simulink model "all_sc_0001_0193"  (R2026a)
settings: Solver=VariableStepAuto  StopTime=40  FixedStep=0.1  MaxStep=.1
model workspace (MAT data in the model file):
  T = [0 0.05 0.1 0.15 0.2 0.25 0.3 0.35 0.4 0.45 0.5 0.55 ... (701 elements, 701x1)]
  U = [3.99594136536 3.99594136536 3.99594136536 3.99594136536 3.99594136536 3.99594136536 3.99594136536 3.99594136536 3.99594136536 3.99594136536 3.99594136536 3.99594136536 ... (701 elements, 701x1)]
undefined symbols (not defined in the file): A, B, C, Dd
(part 2 of 3)

== system all_sc_0001_0193/Subsystem/Steam Condenser1/FIMWB_011 ==
  Original : Inport
  Result : Outport
  wires:
  Original/1 -> Result/1

== system all_sc_0001_0193/Subsystem/Steam Condenser1/FIMWB_012 ==
  Original : Inport
  Result : Outport
  wires:
  Original/1 -> Result/1

== system all_sc_0001_0193/Subsystem/Steam Condenser1/FIMWB_013 ==
  Original : Inport
  Result : Outport
  wires:
  Original/1 -> Result/1

== system all_sc_0001_0193/Subsystem/Steam Condenser1/FIMWB_014 ==
  Original : Inport
  Result : Outport
  wires:
  Original/1 -> Result/1

== system all_sc_0001_0193/Subsystem/Steam Condenser1/FIMWB_015 ==
  Original : Inport
  Result : Outport
  wires:
  Original/1 -> Result/1

== system all_sc_0001_0193/Subsystem/Steam Condenser1/FIMWB_016 ==
  Original : Inport
  Result : Outport
  wires:
  Original/1 -> Result/1

== system all_sc_0001_0193/Subsystem/Steam Condenser1/FIMWB_017 ==
  Original : Inport
  Result : Outport
  wires:
  Original/1 -> Result/1

== system all_sc_0001_0193/Subsystem/Steam Condenser1/FIMWB_018 ==
  Original : Inport
  Result : Outport
  wires:
  Original/1 -> Result/1

== system all_sc_0001_0193/Subsystem/Steam Condenser1/FIMWB_019 ==
  Original : Inport
  Result : Outport
  wires:
  Original/1 -> Result/1

== system all_sc_0001_0193/Subsystem/Steam Condenser1/FIMWB_020 ==
  Original : Inport
  Result : Outport
  wires:
  Original/1 -> Result/1

== system all_sc_0001_0193/Subsystem/Steam Condenser1/FIMWB_021 ==
  Original : Inport
  Result : Outport
  wires:
  Original/1 -> Result/1

== system all_sc_0001_0193/Subsystem/Steam Condenser1/FIMWB_022 ==
  Original : Inport
  Result : Outport
  wires:
  Original/1 -> Result/1

== system all_sc_0001_0193/Subsystem/Steam Condenser1/FIMWB_023 ==
  Original : Inport
  Result : Outport
  wires:
  Original/1 -> Result/1

== system all_sc_0001_0193/Subsystem/Steam Condenser1/FIMWB_024 ==
  Original : Inport
  Result : Outport
  wires:
  Original/1 -> Result/1

== system all_sc_0001_0193/Subsystem/Steam Condenser1/FIMWB_025 ==
  Original : Inport
  Result : Outport
  wires:
  Original/1 -> Result/1

== system all_sc_0001_0193/Subsystem/Steam Condenser1/FIMWB_026 ==
  Original : Inport
  Result : Outport
  wires:
  Original/1 -> Result/1

== system all_sc_0001_0193/Subsystem/Steam Condenser1/FIMWB_027 ==
  Original : Inport
  Result : Outport
  wires:
  Original/1 -> Result/1

== system all_sc_0001_0193/Subsystem/Steam Condenser1/FIMWB_028 ==
  Original : Inport
  Result : Outport
  wires:
  Original/1 -> Result/1

== system all_sc_0001_0193/Subsystem/Steam Condenser1/FIMWB_029 ==
  Original : Inport
  Result : Outport
  wires:
  Original/1 -> Result/1

== system all_sc_0001_0193/Subsystem/Steam Condenser1/FIMWB_030 ==
  Original : Inport
  Result : Outport
  wires:
  Original/1 -> Result/1

== system all_sc_0001_0193/Subsystem/Steam Condenser1/FIMWB_031 ==
  Original : Inport
  Result : Outport
  wires:
  Original/1 -> Result/1

== system all_sc_0001_0193/Subsystem/Steam Condenser1/FIMWB_032 ==
  Original : Inport
  Result : Outport
  wires:
  Original/1 -> Result/1

== system all_sc_0001_0193/Subsystem/Steam Condenser1/FIMWB_033 ==
  Original : Inport
  Result : Outport
  wires:
  Original/1 -> Result/1

== system all_sc_0001_0193/Subsystem/Steam Condenser1/FIMWB_034 ==
  Original : Inport
  Result : Outport
  wires:
  Original/1 -> Result/1

== system all_sc_0001_0193/Subsystem/Steam Condenser1/FIMWB_035 ==
  Original : Inport
  Result : Outport
  wires:
  Original/1 -> Result/1

== system all_sc_0001_0193/Subsystem/Steam Condenser1/FIMWB_036 ==
  Original : Inport
  Result : Outport
  wires:
  Original/1 -> Result/1

== system all_sc_0001_0193/Subsystem/Steam Condenser1/FIMWB_037 ==
  Original : Inport
  Result : Outport
  wires:
  Original/1 -> Result/1

== system all_sc_0001_0193/Subsystem/Steam Condenser1/FIMWB_038 ==
  Original : Inport
  Result : Outport
  wires:
  Original/1 -> Result/1

== system all_sc_0001_0193/Subsystem/Steam Condenser1/FIMWB_039 ==
  Original : Inport
  Result : Outport
  wires:
  Original/1 -> Result/1

== system all_sc_0001_0193/Subsystem/Steam Condenser1/FIMWB_040 ==
  Original : Inport
  Result : Outport
  wires:
  Original/1 -> Result/1

== system all_sc_0001_0193/Subsystem/Steam Condenser1/FIMWB_041 ==
  Original : Inport
  Result : Outport
  wires:
  Original/1 -> Result/1

== system all_sc_0001_0193/Subsystem/Steam Condenser1/FIMWB_044 ==
  Original : Inport
  Result : Outport
  wires:
  Original/1 -> Result/1

== system all_sc_0001_0193/Subsystem/Steam Condenser1/FIMWB_169 ==
  Original : Inport
  Operand1 : Inport  Port=2
  Operand2 : Inport  Port=3
  Unused2 : Terminator
  Unused3 : Terminator
  Result : Outport
  wires:
  Original/1 -> Result/1
  Operand1/1 -> Unused2/1
  Operand2/1 -> Unused3/1

== system all_sc_0001_0193/Subsystem/Steam Condenser1/FIMWB_170 ==
  Original : Inport
  Operand1 : Inport  Port=2
  Operand2 : Inport  Port=3
  Unused2 : Terminator
  Unused3 : Terminator
  Result : Outport
  wires:
  Original/1 -> Result/1
  Operand1/1 -> Unused2/1
  Operand2/1 -> Unused3/1

== system all_sc_0001_0193/Subsystem/Steam Condenser1/FIMWB_171 ==
  Original : Inport
  Operand1 : Inport  Port=2
  Operand2 : Inport  Port=3
  Unused2 : Terminator
  Unused3 : Terminator
  Result : Outport
  wires:
  Original/1 -> Result/1
  Operand1/1 -> Unused2/1
  Operand2/1 -> Unused3/1

== system all_sc_0001_0193/Subsystem/Steam Condenser1/FIMWB_172 ==
  Original : Inport
  Operand1 : Inport  Port=2
  Operand2 : Inport  Port=3
  Unused2 : Terminator
  Unused3 : Terminator
  Result : Outport
  wires:
  Original/1 -> Result/1
  Operand1/1 -> Unused2/1
  Operand2/1 -> Unused3/1

== system all_sc_0001_0193/Subsystem/Steam Condenser1/FIMWB_173 ==
  Original : Inport
  Operand1 : Inport  Port=2
  Operand2 : Inport  Port=3
  Unused2 : Terminator
  Unused3 : Terminator
  Result : Outport
  wires:
  Original/1 -> Result/1
  Operand1/1 -> Unused2/1
  Operand2/1 -> Unused3/1

== system all_sc_0001_0193/Subsystem/Steam Condenser1/FIMWB_174 ==
  Original : Inport
  Operand1 : Inport  Port=2
  Operand2 : Inport  Port=3
  Unused2 : Terminator
  Unused3 : Terminator
  Result : Outport
  wires:
  Original/1 -> Result/1
  Operand1/1 -> Unused2/1
  Operand2/1 -> Unused3/1

== system all_sc_0001_0193/Subsystem/Steam Condenser1/FIMWB_175 ==
  Original : Inport
  Operand1 : Inport  Port=2
  Operand2 : Inport  Port=3
  Unused2 : Terminator
  Unused3 : Terminator
  Result : Outport
  wires:
  Original/1 -> Result/1
  Operand1/1 -> Unused2/1
  Operand2/1 -> Unused3/1

== system all_sc_0001_0193/Subsystem/Steam Condenser1/FIMWB_176 ==
  Original : Inport
  Operand1 : Inport  Port=2
  Operand2 : Inport  Port=3
  Unused2 : Terminator
  Unused3 : Terminator
  Result : Outport
  wires:
  Original/1 -> Result/1
  Operand1/1 -> Unused2/1
  Operand2/1 -> Unused3/1

== system all_sc_0001_0193/Subsystem/Steam Condenser1/FIMWB_180 ==
  Original : Inport
  Result : Outport
  wires:
  Original/1 -> Result/1

== system all_sc_0001_0193/Subsystem/Steam Condenser1/FIMWB_181 ==
  Original : Inport
  Result : Outport
  wires:
  Original/1 -> Result/1

== system all_sc_0001_0193/Subsystem/Steam Condenser1/FIMWB_182 ==
  Original : Inport
  Result : Outport
  wires:
  Original/1 -> Result/1

== system all_sc_0001_0193/Subsystem/Steam Condenser1/FIMWB_183 ==
  Original : Inport
  Result : Outport
  wires:
  Original/1 -> Result/1

== system all_sc_0001_0193/Subsystem/Steam Condenser1/FIMWB_184 ==
  Original : Inport
  Result : Outport
  wires:
  Original/1 -> Result/1

== system all_sc_0001_0193/Subsystem/Steam Condenser1/FIMWB_185 ==
  Original : Inport
  Result : Outport
  wires:
  Original/1 -> Result/1

== system all_sc_0001_0193/Subsystem/Steam Condenser1/FIMWB_186 ==
  Original : Inport
  Result : Outport
  wires:
  Original/1 -> Result/1

== system all_sc_0001_0193/Subsystem/Steam Condenser1/sensor ==
  In1 : Inport
  FIMWB_042 : Subsystem  Tag=fimwb.fault.42
  FIMWB_043 : Subsystem  Tag=fimwb.fault.43
  State Space : StateSpace  A=A  B=B  C=C  D=Dd  InitialCondition=X0
  Out1 : Outport  InitialOutput=0  VectorParamsAs1DForOutWhenUnconnected=off
  wires:
  In1/1 -> FIMWB_042/1(Original)
  FIMWB_042/1(Result) -> State Space/1
  State Space/1 -> FIMWB_043/1(Original)
  FIMWB_043/1(Result) -> Out1/1

== system all_sc_0001_0193/Subsystem/Layer Recurrent Neural Network 3 layers /Layer 1/Delays 1 ==
  "p{1}" : Inport  PortDimensions=1
      mask Display: e = 0.06;c1 = [120 230 180]/255;c2 = ([120 230 180]+0)/(256+128);c3 = ([120 230 180]+128)/(256+128);patch([0 1 1 0],[0 0 1 1],c1);patch([0 1 1 1-e 1-e 0+e],[0 0 1 1-e 0+e 0+e],c2);patch([0 0 1 1-e 0+e 0+e],[0 1 1 1-e 1-e 0+e],c3);plot([0 1 1 0 0],[0 0 1 1 0]);
  FIMWB_058 : Subsystem  Tag=fimwb.fault.58
  FIMWB_059 : Subsystem  Tag=fimwb.fault.59
  mux : Mux  Inputs=1
      mask Display: e = 0.06;c1 = [120 150 230]/255;c2 = ([120 150 230]+0)/383;c3 = ([120 150 230]+128)/383;patch([0 1 1 0],[0 0 1 1],c1);patch([0 1 1 1-e 1-e 0+e],[0 0 1 1-e 0+e 0+e],c2);patch([0 0 1 1-e 0+e 0+e],[0 1 1 1-e 1-e 0+e],c3);plot([0 1 1 0 0],[0 0 1 1 0]);disp('Mux')
  "pd{1,1}" : Outport  VectorParamsAs1DForOutWhenUnconnected=off
      mask Display: e = 0.06;c1 = [120 230 180]/255;c2 = ([120 230 180]+0)/(256+128);c3 = ([120 230 180]+128)/(256+128);patch([0 1 1 0],[0 0 1 1],c1);patch([0 1 1 1-e 1-e 0+e],[0 0 1 1-e 0+e 0+e],c2);patch([0 0 1 1-e 0+e 0+e],[0 1 1 1-e 1-e 0+e],c3);plot([0 1 1 0 0],[0 0 1 1 0]);
  wires:
  "p{1}"/1 -> FIMWB_058/1(Original)
  FIMWB_058/1(Result) -> mux/1
  mux/1 -> FIMWB_059/1(Original)
  FIMWB_059/1(Result) -> "pd{1,1}"/1

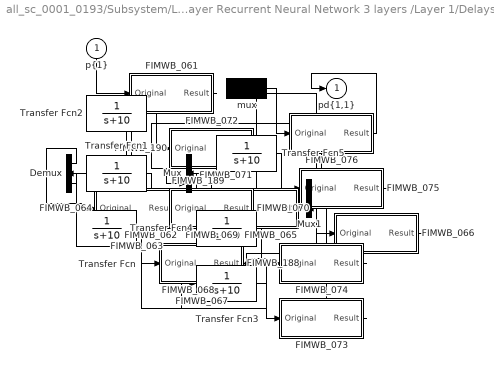
== system all_sc_0001_0193/Subsystem/Layer Recurrent Neural Network 3 layers /Layer 1/Delays 2 ==
  "p{1}" : Inport  PortDimensions=3
      mask Display: e = 0.06;c1 = [120 230 180]/255;c2 = ([120 230 180]+0)/(256+128);c3 = ([120 230 180]+128)/(256+128);patch([0 1 1 0],[0 0 1 1],c1);patch([0 1 1 1-e 1-e 0+e],[0 0 1 1-e 0+e 0+e],c2);patch([0 0 1 1-e 0+e 0+e],[0 1 1 1-e 1-e 0+e],c3);plot([0 1 1 0 0],[0 0 1 1 0]);
  Demux : Demux  Outputs=3
  FIMWB_061 : Subsystem  Tag=fimwb.fault.61
  FIMWB_062 : Subsystem  Tag=fimwb.fault.62
  FIMWB_063 : Subsystem  Tag=fimwb.fault.63
  FIMWB_064 : Subsystem  Tag=fimwb.fault.64
  FIMWB_065 : Subsystem  Tag=fimwb.fault.65
  FIMWB_066 : Subsystem  Tag=fimwb.fault.66
  FIMWB_067 : Subsystem  Tag=fimwb.fault.67
  FIMWB_068 : Subsystem  Tag=fimwb.fault.68
  FIMWB_069 : Subsystem  Tag=fimwb.fault.69
  FIMWB_070 : Subsystem  Tag=fimwb.fault.70
  FIMWB_071 : Subsystem  Tag=fimwb.fault.71
  FIMWB_072 : Subsystem  Tag=fimwb.fault.72
  FIMWB_073 : Subsystem  Tag=fimwb.fault.73
  FIMWB_074 : Subsystem  Tag=fimwb.fault.74
  FIMWB_075 : Subsystem  Tag=fimwb.fault.75
  FIMWB_076 : Subsystem  Tag=fimwb.fault.76
  FIMWB_188 : Subsystem  Tag=fimwb.fault.188
  FIMWB_189 : Subsystem  Tag=fimwb.fault.189
  FIMWB_190 : Subsystem  Tag=fimwb.fault.190
  Mux : Mux  Inputs=3
  Mux1 : Mux  Inputs=3
  Transfer Fcn{,1..5} (6 alike) : TransferFcn  Denominator=[1 10]
  mux : Mux  Inputs=2
      mask Display: e = 0.06;c1 = [120 150 230]/255;c2 = ([120 150 230]+0)/383;c3 = ([120 150 230]+128)/383;patch([0 1 1 0],[0 0 1 1],c1);patch([0 1 1 1-e 1-e 0+e],[0 0 1 1-e 0+e 0+e],c2);patch([0 0 1 1-e 0+e 0+e],[0 1 1 1-e 1-e 0+e],c3);plot([0 1 1 0 0],[0 0 1 1 0]);disp('Mux')
  "pd{1,1}" : Outport  VectorParamsAs1DForOutWhenUnconnected=off
      mask Display: e = 0.06;c1 = [120 230 180]/255;c2 = ([120 230 180]+0)/(256+128);c3 = ([120 230 180]+128)/(256+128);patch([0 1 1 0],[0 0 1 1],c1);patch([0 1 1 1-e 1-e 0+e],[0 0 1 1-e 0+e 0+e],c2);patch([0 0 1 1-e 0+e 0+e],[0 1 1 1-e 1-e 0+e],c3);plot([0 1 1 0 0],[0 0 1 1 0]);
  wires:
  Transfer Fcn/1 -> FIMWB_188/1(Original)
  FIMWB_188/1(Result) -> FIMWB_067/1(Original), FIMWB_068/1(Original)
  Transfer Fcn1/1 -> FIMWB_189/1(Original)
  FIMWB_189/1(Result) -> FIMWB_069/1(Original), FIMWB_070/1(Original)
  Transfer Fcn2/1 -> FIMWB_190/1(Original)
  FIMWB_190/1(Result) -> FIMWB_071/1(Original), FIMWB_072/1(Original)
  "p{1}"/1 -> FIMWB_061/1(Original)
  FIMWB_061/1(Result) -> Demux/1
  Demux/1 -> FIMWB_062/1(Original)
  FIMWB_062/1(Result) -> Transfer Fcn2/1
  Demux/2 -> FIMWB_063/1(Original)
  FIMWB_063/1(Result) -> Transfer Fcn1/1
  Demux/3 -> FIMWB_064/1(Original)
  FIMWB_064/1(Result) -> Transfer Fcn/1
  Mux/1 -> FIMWB_065/1(Original)
  FIMWB_065/1(Result) -> mux/1
  Mux1/1 -> FIMWB_066/1(Original)
  FIMWB_066/1(Result) -> mux/2
  FIMWB_067/1(Result) -> Mux/3
  FIMWB_068/1(Result) -> Transfer Fcn3/1
  FIMWB_069/1(Result) -> Mux/2
  FIMWB_070/1(Result) -> Transfer Fcn4/1
  FIMWB_071/1(Result) -> Mux/1
  FIMWB_072/1(Result) -> Transfer Fcn5/1
  Transfer Fcn3/1 -> FIMWB_073/1(Original)
  FIMWB_073/1(Result) -> Mux1/3
  Transfer Fcn4/1 -> FIMWB_074/1(Original)
  FIMWB_074/1(Result) -> Mux1/2
  Transfer Fcn5/1 -> FIMWB_075/1(Original)
  FIMWB_075/1(Result) -> Mux1/1
  mux/1 -> FIMWB_076/1(Original)
  FIMWB_076/1(Result) -> "pd{1,1}"/1

== system all_sc_0001_0193/Subsystem/Layer Recurrent Neural Network 3 layers /Layer 1/FIMWB_055 ==
  Original : Inport
  Result : Outport
  wires:
  Original/1 -> Result/1

== system all_sc_0001_0193/Subsystem/Layer Recurrent Neural Network 3 layers /Layer 1/FIMWB_056 ==
  Original : Inport
  Result : Outport
  wires:
  Original/1 -> Result/1

== system all_sc_0001_0193/Subsystem/Layer Recurrent Neural Network 3 layers /Layer 1/FIMWB_057 ==
  Original : Inport
  Result : Outport
  wires:
  Original/1 -> Result/1

== system all_sc_0001_0193/Subsystem/Layer Recurrent Neural Network 3 layers /Layer 1/FIMWB_060 ==
  Original : Inport
  Result : Outport
  wires:
  Original/1 -> Result/1

== system all_sc_0001_0193/Subsystem/Layer Recurrent Neural Network 3 layers /Layer 1/FIMWB_077 ==
  Original : Inport
  Result : Outport
  wires:
  Original/1 -> Result/1

== system all_sc_0001_0193/Subsystem/Layer Recurrent Neural Network 3 layers /Layer 1/FIMWB_097 ==
  Original : Inport
  Result : Outport
  wires:
  Original/1 -> Result/1

== system all_sc_0001_0193/Subsystem/Layer Recurrent Neural Network 3 layers /Layer 1/FIMWB_117 ==
  Original : Inport
  Result : Outport
  wires:
  Original/1 -> Result/1

== system all_sc_0001_0193/Subsystem/Layer Recurrent Neural Network 3 layers /Layer 1/FIMWB_118 ==
  Original : Inport
  Result : Outport
  wires:
  Original/1 -> Result/1

== system all_sc_0001_0193/Subsystem/Layer Recurrent Neural Network 3 layers /Layer 1/FIMWB_128 ==
  Original : Inport
  Result : Outport
  wires:
  Original/1 -> Result/1

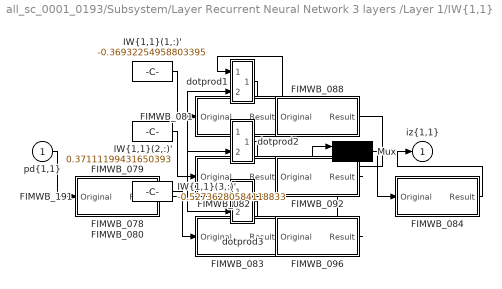
== system all_sc_0001_0193/Subsystem/Layer Recurrent Neural Network 3 layers /Layer 1/IW{1,1} ==
  "pd{1,1}" : Inport  PortDimensions=1
      mask Display: e = 0.06;c1 = [120 230 180]/255;c2 = ([120 230 180]+0)/(256+128);c3 = ([120 230 180]+128)/(256+128);patch([0 1 1 0],[0 0 1 1],c1);patch([0 1 1 1-e 1-e 0+e],[0 0 1 1-e 0+e 0+e],c2);patch([0 0 1 1-e 0+e 0+e],[0 1 1 1-e 1-e 0+e],c3);plot([0 1 1 0 0],[0 0 1 1 0]);
  FIMWB_078 : Subsystem  Tag=fimwb.fault.78
  FIMWB_079 : Subsystem  Tag=fimwb.fault.79
  FIMWB_080 : Subsystem  Tag=fimwb.fault.80
  FIMWB_081 : Subsystem  Tag=fimwb.fault.81
  FIMWB_082 : Subsystem  Tag=fimwb.fault.82
  FIMWB_083 : Subsystem  Tag=fimwb.fault.83
  FIMWB_084 : Subsystem  Tag=fimwb.fault.84
  FIMWB_088 : Subsystem  Tag=fimwb.fault.88
  FIMWB_092 : Subsystem  Tag=fimwb.fault.92
  FIMWB_096 : Subsystem  Tag=fimwb.fault.96
  FIMWB_191 : Subsystem  Tag=fimwb.fault.191
  "IW{1,1}(1,:)'" : Constant  Value=-0.36932254958803395
      mask Display: e = 0.06;c1 = [120 150 230]/255;c2 = ([120 150 230]+0)/383;c3 = ([120 150 230]+128)/383;patch([0 1 1 0],[0 0 1 1],c1);patch([0 1 1 1-e 1-e 0+e],[0 0 1 1-e 0+e 0+e],c2);patch([0 0 1 1-e 0+e 0+e],[0 1 1 1-e 1-e 0+e],c3);plot([0 1 1 0 0],[0 0 1 1 0]);disp('Weights');
  "IW{1,1}(2,:)'" : Constant  Value=0.37111199431650393
      mask Display: e = 0.06;c1 = [120 150 230]/255;c2 = ([120 150 230]+0)/383;c3 = ([120 150 230]+128)/383;patch([0 1 1 0],[0 0 1 1],c1);patch([0 1 1 1-e 1-e 0+e],[0 0 1 1-e 0+e 0+e],c2);patch([0 0 1 1-e 0+e 0+e],[0 1 1 1-e 1-e 0+e],c3);plot([0 1 1 0 0],[0 0 1 1 0]);disp('Weights');
  "IW{1,1}(3,:)'" : Constant  Value=-0.52736280584118833
      mask Display: e = 0.06;c1 = [120 150 230]/255;c2 = ([120 150 230]+0)/383;c3 = ([120 150 230]+128)/383;patch([0 1 1 0],[0 0 1 1],c1);patch([0 1 1 1-e 1-e 0+e],[0 0 1 1-e 0+e 0+e],c2);patch([0 0 1 1-e 0+e 0+e],[0 1 1 1-e 1-e 0+e],c3);plot([0 1 1 0 0],[0 0 1 1 0]);disp('Weights');
  Mux : Mux  Inputs=3
      mask Display: e = 0.06;c1 = [120 150 230]/255;c2 = ([120 150 230]+0)/383;c3 = ([120 150 230]+128)/383;patch([0 1 1 0],[0 0 1 1],c1);patch([0 1 1 1-e 1-e 0+e],[0 0 1 1-e 0+e 0+e],c2);patch([0 0 1 1-e 0+e 0+e],[0 1 1 1-e 1-e 0+e],c3);plot([0 1 1 0 0],[0 0 1 1 0]);disp('Mux');
  dotprod1 : Subsystem  mask(DOTPROD){}
      mask help: nnet:Simulink:DotprodBlockDesc
      mask init:
      | network;
      mask Help: helpview([docroot '/deeplearning/ref/dotprod.html']);
      mask Display:
      | e = 0.06;
      | c1 = [120 150 230]/255;
      | c2 = ([120 150 230]+0)/383;
      | c3 = ([120 150 230]+128)/383;
      | patch([0 1 1 0],[0 0 1 1],c1);
      | patch([0 1 1 1-e 1-e 0+e],[0 0 1 1-e 0+e 0+e],c2);
      | patch([0 0 1 1-e 0+e 0+e],[0 1 1 1-e 1-e 0+e],c3);
      | plot([0 1 1 0 0],[0 0 1 1 0])
      | port_label('input',1,'w')
      | port_label('input',2,'p')
      | port_label('output',1,'z')
  dotprod2 : Subsystem  mask(DOTPROD){}
      mask help: nnet:Simulink:DotprodBlockDesc
      mask init:
      | network;
      mask Help: helpview([docroot '/deeplearning/ref/dotprod.html']);
      mask Display:
      | e = 0.06;
      | c1 = [120 150 230]/255;
      | c2 = ([120 150 230]+0)/383;
      | c3 = ([120 150 230]+128)/383;
      | patch([0 1 1 0],[0 0 1 1],c1);
      | patch([0 1 1 1-e 1-e 0+e],[0 0 1 1-e 0+e 0+e],c2);
      | patch([0 0 1 1-e 0+e 0+e],[0 1 1 1-e 1-e 0+e],c3);
      | plot([0 1 1 0 0],[0 0 1 1 0])
      | port_label('input',1,'w')
      | port_label('input',2,'p')
      | port_label('output',1,'z')
  dotprod3 : Subsystem  mask(DOTPROD){}
      mask help: nnet:Simulink:DotprodBlockDesc
      mask init:
      | network;
      mask Help: helpview([docroot '/deeplearning/ref/dotprod.html']);
      mask Display:
      | e = 0.06;
      | c1 = [120 150 230]/255;
      | c2 = ([120 150 230]+0)/383;
      | c3 = ([120 150 230]+128)/383;
      | patch([0 1 1 0],[0 0 1 1],c1);
      | patch([0 1 1 1-e 1-e 0+e],[0 0 1 1-e 0+e 0+e],c2);
      | patch([0 0 1 1-e 0+e 0+e],[0 1 1 1-e 1-e 0+e],c3);
      | plot([0 1 1 0 0],[0 0 1 1 0])
      | port_label('input',1,'w')
      | port_label('input',2,'p')
      | port_label('output',1,'z')
  "iz{1,1}" : Outport  VectorParamsAs1DForOutWhenUnconnected=off
      mask Display: e = 0.06;c1 = [120 230 180]/255;c2 = ([120 230 180]+0)/(256+128);c3 = ([120 230 180]+128)/(256+128);patch([0 1 1 0],[0 0 1 1],c1);patch([0 1 1 1-e 1-e 0+e],[0 0 1 1-e 0+e 0+e],c2);patch([0 0 1 1-e 0+e 0+e],[0 1 1 1-e 1-e 0+e],c3);plot([0 1 1 0 0],[0 0 1 1 0]);
  wires:
  "pd{1,1}"/1 -> FIMWB_191/1(Original)
  FIMWB_191/1(Result) -> FIMWB_078/1(Original), FIMWB_079/1(Original), FIMWB_080/1(Original)
  FIMWB_078/1(Result) -> dotprod1/2(In2)
  FIMWB_079/1(Result) -> dotprod2/2(In2)
  FIMWB_080/1(Result) -> dotprod3/2(In2)
  "IW{1,1}(1,:)'"/1 -> FIMWB_081/1(Original)
  FIMWB_081/1(Result) -> dotprod1/1(In1)
  "IW{1,1}(2,:)'"/1 -> FIMWB_082/1(Original)
  FIMWB_082/1(Result) -> dotprod2/1(In1)
  "IW{1,1}(3,:)'"/1 -> FIMWB_083/1(Original)
  FIMWB_083/1(Result) -> dotprod3/1(In1)
  Mux/1 -> FIMWB_084/1(Original)
  FIMWB_084/1(Result) -> "iz{1,1}"/1
  dotprod1/1(Out1) -> FIMWB_088/1(Original)
  FIMWB_088/1(Result) -> Mux/1
  dotprod2/1(Out1) -> FIMWB_092/1(Original)
  FIMWB_092/1(Result) -> Mux/2
  dotprod3/1(Out1) -> FIMWB_096/1(Original)
  FIMWB_096/1(Result) -> Mux/3

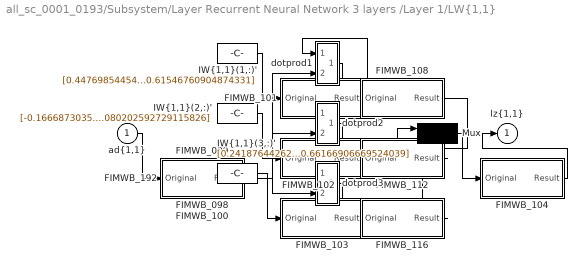
== system all_sc_0001_0193/Subsystem/Layer Recurrent Neural Network 3 layers /Layer 1/LW{1,1} ==
  "ad{1,1}" : Inport  PortDimensions=6
      mask Display: e = 0.06;c1 = [120 230 180]/255;c2 = ([120 230 180]+0)/(256+128);c3 = ([120 230 180]+128)/(256+128);patch([0 1 1 0],[0 0 1 1],c1);patch([0 1 1 1-e 1-e 0+e],[0 0 1 1-e 0+e 0+e],c2);patch([0 0 1 1-e 0+e 0+e],[0 1 1 1-e 1-e 0+e],c3);plot([0 1 1 0 0],[0 0 1 1 0]);
  FIMWB_098 : Subsystem  Tag=fimwb.fault.98
  FIMWB_099 : Subsystem  Tag=fimwb.fault.99
  FIMWB_100 : Subsystem  Tag=fimwb.fault.100
  FIMWB_101 : Subsystem  Tag=fimwb.fault.101
  FIMWB_102 : Subsystem  Tag=fimwb.fault.102
  FIMWB_103 : Subsystem  Tag=fimwb.fault.103
  FIMWB_104 : Subsystem  Tag=fimwb.fault.104
  FIMWB_108 : Subsystem  Tag=fimwb.fault.108
  FIMWB_112 : Subsystem  Tag=fimwb.fault.112
  FIMWB_116 : Subsystem  Tag=fimwb.fault.116
  FIMWB_192 : Subsystem  Tag=fimwb.fault.192
  "IW{1,1}(1,:)'" : Constant  Value=[0.44769854454577174;1.1961840315574388;1.1412233787458486;0.72001623019786209;-0.37547125154051064;-0.61546760904874331]
      mask Display: e = 0.06;c1 = [120 150 230]/255;c2 = ([120 150 230]+0)/383;c3 = ([120 150 230]+128)/383;patch([0 1 1 0],[0 0 1 1],c1);patch([0 1 1 1-e 1-e 0+e],[0 0 1 1-e 0+e 0+e],c2);patch([0 0 1 1-e 0+e 0+e],[0 1 1 1-e 1-e 0+e],c3);plot([0 1 1 0 0],[0 0 1 1 0]);disp('weights');
  "IW{1,1}(2,:)'" : Constant  Value=[-0.16668730359454359;-0.016432941671533533;-0.22132796342367161;-0.037206224095552992;0.059874671921603305;0.080202592729115826]
      mask Display: e = 0.06;c1 = [120 150 230]/255;c2 = ([120 150 230]+0)/383;c3 = ([120 150 230]+128)/383;patch([0 1 1 0],[0 0 1 1],c1);patch([0 1 1 1-e 1-e 0+e],[0 0 1 1-e 0+e 0+e],c2);patch([0 0 1 1-e 0+e 0+e],[0 1 1 1-e 1-e 0+e],c3);plot([0 1 1 0 0],[0 0 1 1 0]);disp('weights');
  "IW{1,1}(3,:)'" : Constant  Value=[0.24187644262601646;-0.66963285238228187;-1.0984401489322673;0.029109804692608397;1.3722216833345802;0.66166906669524039]
      mask Display: e = 0.06;c1 = [120 150 230]/255;c2 = ([120 150 230]+0)/383;c3 = ([120 150 230]+128)/383;patch([0 1 1 0],[0 0 1 1],c1);patch([0 1 1 1-e 1-e 0+e],[0 0 1 1-e 0+e 0+e],c2);patch([0 0 1 1-e 0+e 0+e],[0 1 1 1-e 1-e 0+e],c3);plot([0 1 1 0 0],[0 0 1 1 0]);disp('weights');
  Mux : Mux  Inputs=3
      mask Display: e = 0.06;c1 = [120 150 230]/255;c2 = ([120 150 230]+0)/383;c3 = ([120 150 230]+128)/383;patch([0 1 1 0],[0 0 1 1],c1);patch([0 1 1 1-e 1-e 0+e],[0 0 1 1-e 0+e 0+e],c2);patch([0 0 1 1-e 0+e 0+e],[0 1 1 1-e 1-e 0+e],c3);plot([0 1 1 0 0],[0 0 1 1 0]);disp('Mux');
  dotprod1 : Subsystem  mask(DOTPROD){}
      mask help: nnet:Simulink:DotprodBlockDesc
      mask init:
      | network;
      mask Help: helpview([docroot '/deeplearning/ref/dotprod.html']);
      mask Display:
      | e = 0.06;
      | c1 = [120 150 230]/255;
      | c2 = ([120 150 230]+0)/383;
      | c3 = ([120 150 230]+128)/383;
      | patch([0 1 1 0],[0 0 1 1],c1);
      | patch([0 1 1 1-e 1-e 0+e],[0 0 1 1-e 0+e 0+e],c2);
      | patch([0 0 1 1-e 0+e 0+e],[0 1 1 1-e 1-e 0+e],c3);
      | plot([0 1 1 0 0],[0 0 1 1 0])
      | port_label('input',1,'w')
      | port_label('input',2,'p')
      | port_label('output',1,'z')
  dotprod2 : Subsystem  mask(DOTPROD){}
      mask help: nnet:Simulink:DotprodBlockDesc
      mask init:
      | network;
      mask Help: helpview([docroot '/deeplearning/ref/dotprod.html']);
      mask Display:
      | e = 0.06;
      | c1 = [120 150 230]/255;
      | c2 = ([120 150 230]+0)/383;
      | c3 = ([120 150 230]+128)/383;
      | patch([0 1 1 0],[0 0 1 1],c1);
      | patch([0 1 1 1-e 1-e 0+e],[0 0 1 1-e 0+e 0+e],c2);
      | patch([0 0 1 1-e 0+e 0+e],[0 1 1 1-e 1-e 0+e],c3);
      | plot([0 1 1 0 0],[0 0 1 1 0])
      | port_label('input',1,'w')
      | port_label('input',2,'p')
      | port_label('output',1,'z')
  dotprod3 : Subsystem  mask(DOTPROD){}
      mask help: nnet:Simulink:DotprodBlockDesc
      mask init:
      | network;
      mask Help: helpview([docroot '/deeplearning/ref/dotprod.html']);
      mask Display:
      | e = 0.06;
      | c1 = [120 150 230]/255;
      | c2 = ([120 150 230]+0)/383;
      | c3 = ([120 150 230]+128)/383;
      | patch([0 1 1 0],[0 0 1 1],c1);
      | patch([0 1 1 1-e 1-e 0+e],[0 0 1 1-e 0+e 0+e],c2);
      | patch([0 0 1 1-e 0+e 0+e],[0 1 1 1-e 1-e 0+e],c3);
      | plot([0 1 1 0 0],[0 0 1 1 0])
      | port_label('input',1,'w')
      | port_label('input',2,'p')
      | port_label('output',1,'z')
  "lz{1,1}" : Outport  VectorParamsAs1DForOutWhenUnconnected=off
      mask Display: e = 0.06;c1 = [120 230 180]/255;c2 = ([120 230 180]+0)/(256+128);c3 = ([120 230 180]+128)/(256+128);patch([0 1 1 0],[0 0 1 1],c1);patch([0 1 1 1-e 1-e 0+e],[0 0 1 1-e 0+e 0+e],c2);patch([0 0 1 1-e 0+e 0+e],[0 1 1 1-e 1-e 0+e],c3);plot([0 1 1 0 0],[0 0 1 1 0]);
  wires:
  "ad{1,1}"/1 -> FIMWB_192/1(Original)
  FIMWB_192/1(Result) -> FIMWB_098/1(Original), FIMWB_099/1(Original), FIMWB_100/1(Original)
  FIMWB_098/1(Result) -> dotprod1/2(In2)
  FIMWB_099/1(Result) -> dotprod2/2(In2)
  FIMWB_100/1(Result) -> dotprod3/2(In2)
  "IW{1,1}(1,:)'"/1 -> FIMWB_101/1(Original)
  FIMWB_101/1(Result) -> dotprod1/1(In1)
  "IW{1,1}(2,:)'"/1 -> FIMWB_102/1(Original)
  FIMWB_102/1(Result) -> dotprod2/1(In1)
  "IW{1,1}(3,:)'"/1 -> FIMWB_103/1(Original)
  FIMWB_103/1(Result) -> dotprod3/1(In1)
  Mux/1 -> FIMWB_104/1(Original)
  FIMWB_104/1(Result) -> "lz{1,1}"/1
  dotprod1/1(Out1) -> FIMWB_108/1(Original)
  FIMWB_108/1(Result) -> Mux/1
  dotprod2/1(Out1) -> FIMWB_112/1(Original)
  FIMWB_112/1(Result) -> Mux/2
  dotprod3/1(Out1) -> FIMWB_116/1(Original)
  FIMWB_116/1(Result) -> Mux/3

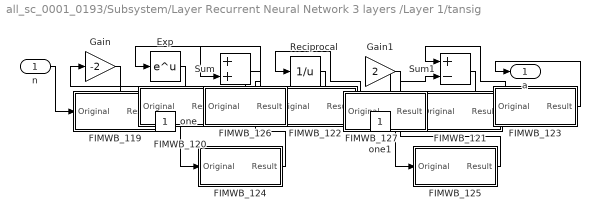
== system all_sc_0001_0193/Subsystem/Layer Recurrent Neural Network 3 layers /Layer 1/tansig ==
  n : Inport
  Exp : Math  SignedPower=on
  FIMWB_119 : Subsystem  Tag=fimwb.fault.119
  FIMWB_120 : Subsystem  Tag=fimwb.fault.120
  FIMWB_121 : Subsystem  Tag=fimwb.fault.121
  FIMWB_122 : Subsystem  Tag=fimwb.fault.122
  FIMWB_123 : Subsystem  Tag=fimwb.fault.123
  FIMWB_124 : Subsystem  Tag=fimwb.fault.124
  FIMWB_125 : Subsystem  Tag=fimwb.fault.125
  FIMWB_126 : Subsystem  Tag=fimwb.fault.126
  FIMWB_127 : Subsystem  Tag=fimwb.fault.127
  Gain : Gain  Gain=-2  SaturateOnIntegerOverflow=on  OutDataTypeStr=Inherit: Same as input  ParamDataTypeStr=Inherit: Same as input
  Gain1 : Gain  Gain=2  SaturateOnIntegerOverflow=on  OutDataTypeStr=Inherit: Same as input  ParamDataTypeStr=Inherit: Same as input
  Reciprocal : Math  Operator=reciprocal  SignedPower=on
  Sum : Sum  InputSameDT=on  SaturateOnIntegerOverflow=on  OutDataTypeStr=Inherit: Same as first input
  Sum1 : Sum  Inputs=+-  InputSameDT=on  SaturateOnIntegerOverflow=on  OutDataTypeStr=Inherit: Same as first input
  one : Constant
  one1 : Constant
  a : Outport  InitialOutput=0  VectorParamsAs1DForOutWhenUnconnected=off
  wires:
  n/1 -> FIMWB_119/1(Original)
  FIMWB_119/1(Result) -> Gain/1
  Gain/1 -> FIMWB_120/1(Original)
  FIMWB_120/1(Result) -> Exp/1
  Gain1/1 -> FIMWB_121/1(Original)
  FIMWB_121/1(Result) -> Sum1/1
  Sum/1 -> FIMWB_122/1(Original)
  FIMWB_122/1(Result) -> Reciprocal/1
  Sum1/1 -> FIMWB_123/1(Original)
  FIMWB_123/1(Result) -> a/1
  one/1 -> FIMWB_124/1(Original)
  FIMWB_124/1(Result) -> Sum/2
  one1/1 -> FIMWB_125/1(Original)
  FIMWB_125/1(Result) -> Sum1/2
  Exp/1 -> FIMWB_126/1(Original)
  FIMWB_126/1(Result) -> Sum/1
  Reciprocal/1 -> FIMWB_127/1(Original)
  FIMWB_127/1(Result) -> Gain1/1

== system all_sc_0001_0193/Subsystem/Layer Recurrent Neural Network 3 layers /Layer 2/Delays 1 ==
  "p{2}" : Inport  PortDimensions=3
      mask Display: e = 0.06;c1 = [120 230 180]/255;c2 = ([120 230 180]+0)/(256+128);c3 = ([120 230 180]+128)/(256+128);patch([0 1 1 0],[0 0 1 1],c1);patch([0 1 1 1-e 1-e 0+e],[0 0 1 1-e 0+e 0+e],c2);patch([0 0 1 1-e 0+e 0+e],[0 1 1 1-e 1-e 0+e],c3);plot([0 1 1 0 0],[0 0 1 1 0]);
  FIMWB_132 : Subsystem  Tag=fimwb.fault.132
  FIMWB_133 : Subsystem  Tag=fimwb.fault.133
  mux : Mux  Inputs=1
      mask Display: e = 0.06;c1 = [120 150 230]/255;c2 = ([120 150 230]+0)/383;c3 = ([120 150 230]+128)/383;patch([0 1 1 0],[0 0 1 1],c1);patch([0 1 1 1-e 1-e 0+e],[0 0 1 1-e 0+e 0+e],c2);patch([0 0 1 1-e 0+e 0+e],[0 1 1 1-e 1-e 0+e],c3);plot([0 1 1 0 0],[0 0 1 1 0]);disp('Mux')
  "pd{2,1}" : Outport  VectorParamsAs1DForOutWhenUnconnected=off
      mask Display: e = 0.06;c1 = [120 230 180]/255;c2 = ([120 230 180]+0)/(256+128);c3 = ([120 230 180]+128)/(256+128);patch([0 1 1 0],[0 0 1 1],c1);patch([0 1 1 1-e 1-e 0+e],[0 0 1 1-e 0+e 0+e],c2);patch([0 0 1 1-e 0+e 0+e],[0 1 1 1-e 1-e 0+e],c3);plot([0 1 1 0 0],[0 0 1 1 0]);
  wires:
  "p{2}"/1 -> FIMWB_132/1(Original)
  FIMWB_132/1(Result) -> mux/1
  mux/1 -> FIMWB_133/1(Original)
  FIMWB_133/1(Result) -> "pd{2,1}"/1

== system all_sc_0001_0193/Subsystem/Layer Recurrent Neural Network 3 layers /Layer 2/FIMWB_130 ==
  Original : Inport
  Result : Outport
  wires:
  Original/1 -> Result/1

== system all_sc_0001_0193/Subsystem/Layer Recurrent Neural Network 3 layers /Layer 2/FIMWB_131 ==
  Original : Inport
  Result : Outport
  wires:
  Original/1 -> Result/1

== system all_sc_0001_0193/Subsystem/Layer Recurrent Neural Network 3 layers /Layer 2/FIMWB_134 ==
  Original : Inport
  Result : Outport
  wires:
  Original/1 -> Result/1

== system all_sc_0001_0193/Subsystem/Layer Recurrent Neural Network 3 layers /Layer 2/FIMWB_142 ==
  Original : Inport
  Result : Outport
  wires:
  Original/1 -> Result/1

== system all_sc_0001_0193/Subsystem/Layer Recurrent Neural Network 3 layers /Layer 2/FIMWB_143 ==
  Original : Inport
  Result : Outport
  wires:
  Original/1 -> Result/1

== system all_sc_0001_0193/Subsystem/Layer Recurrent Neural Network 3 layers /Layer 2/FIMWB_145 ==
  Original : Inport
  Result : Outport
  wires:
  Original/1 -> Result/1

== system all_sc_0001_0193/Subsystem/Layer Recurrent Neural Network 3 layers /Layer 2/FIMWB_179 ==
  Original : Inport
  Operand1 : Inport  Port=2
  Operand2 : Inport  Port=3
  Unused2 : Terminator
  Unused3 : Terminator
  Result : Outport
  wires:
  Original/1 -> Result/1
  Operand1/1 -> Unused2/1
  Operand2/1 -> Unused3/1

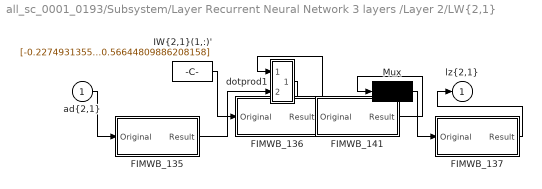
== system all_sc_0001_0193/Subsystem/Layer Recurrent Neural Network 3 layers /Layer 2/LW{2,1} ==
  "ad{2,1}" : Inport  PortDimensions=3
      mask Display: e = 0.06;c1 = [120 230 180]/255;c2 = ([120 230 180]+0)/(256+128);c3 = ([120 230 180]+128)/(256+128);patch([0 1 1 0],[0 0 1 1],c1);patch([0 1 1 1-e 1-e 0+e],[0 0 1 1-e 0+e 0+e],c2);patch([0 0 1 1-e 0+e 0+e],[0 1 1 1-e 1-e 0+e],c3);plot([0 1 1 0 0],[0 0 1 1 0]);
  FIMWB_135 : Subsystem  Tag=fimwb.fault.135
  FIMWB_136 : Subsystem  Tag=fimwb.fault.136
  FIMWB_137 : Subsystem  Tag=fimwb.fault.137
  FIMWB_141 : Subsystem  Tag=fimwb.fault.141
  "IW{2,1}(1,:)'" : Constant  Value=[-0.22749313555095124;2.0804967759906643;-0.56644809886208158]
      mask Display: e = 0.06;c1 = [120 150 230]/255;c2 = ([120 150 230]+0)/383;c3 = ([120 150 230]+128)/383;patch([0 1 1 0],[0 0 1 1],c1);patch([0 1 1 1-e 1-e 0+e],[0 0 1 1-e 0+e 0+e],c2);patch([0 0 1 1-e 0+e 0+e],[0 1 1 1-e 1-e 0+e],c3);plot([0 1 1 0 0],[0 0 1 1 0]);disp('weights');
  Mux : Mux  Inputs=1
      mask Display: e = 0.06;c1 = [120 150 230]/255;c2 = ([120 150 230]+0)/383;c3 = ([120 150 230]+128)/383;patch([0 1 1 0],[0 0 1 1],c1);patch([0 1 1 1-e 1-e 0+e],[0 0 1 1-e 0+e 0+e],c2);patch([0 0 1 1-e 0+e 0+e],[0 1 1 1-e 1-e 0+e],c3);plot([0 1 1 0 0],[0 0 1 1 0]);disp('Mux');
  dotprod1 : Subsystem  mask(DOTPROD){}
      mask help: nnet:Simulink:DotprodBlockDesc
      mask init:
      | network;
      mask Help: helpview([docroot '/deeplearning/ref/dotprod.html']);
      mask Display:
      | e = 0.06;
      | c1 = [120 150 230]/255;
      | c2 = ([120 150 230]+0)/383;
      | c3 = ([120 150 230]+128)/383;
      | patch([0 1 1 0],[0 0 1 1],c1);
      | patch([0 1 1 1-e 1-e 0+e],[0 0 1 1-e 0+e 0+e],c2);
      | patch([0 0 1 1-e 0+e 0+e],[0 1 1 1-e 1-e 0+e],c3);
      | plot([0 1 1 0 0],[0 0 1 1 0])
      | port_label('input',1,'w')
      | port_label('input',2,'p')
      | port_label('output',1,'z')
  "lz{2,1}" : Outport  VectorParamsAs1DForOutWhenUnconnected=off
      mask Display: e = 0.06;c1 = [120 230 180]/255;c2 = ([120 230 180]+0)/(256+128);c3 = ([120 230 180]+128)/(256+128);patch([0 1 1 0],[0 0 1 1],c1);patch([0 1 1 1-e 1-e 0+e],[0 0 1 1-e 0+e 0+e],c2);patch([0 0 1 1-e 0+e 0+e],[0 1 1 1-e 1-e 0+e],c3);plot([0 1 1 0 0],[0 0 1 1 0]);
  wires:
  "ad{2,1}"/1 -> FIMWB_135/1(Original)
  FIMWB_135/1(Result) -> dotprod1/2(In2)
  "IW{2,1}(1,:)'"/1 -> FIMWB_136/1(Original)
  FIMWB_136/1(Result) -> dotprod1/1(In1)
  Mux/1 -> FIMWB_137/1(Original)
  FIMWB_137/1(Result) -> "lz{2,1}"/1
  dotprod1/1(Out1) -> FIMWB_141/1(Original)
  FIMWB_141/1(Result) -> Mux/1

== system all_sc_0001_0193/Subsystem/Layer Recurrent Neural Network 3 layers /Layer 2/purelin ==
  n : Inport
  FIMWB_144 : Subsystem  Tag=fimwb.fault.144
  a : Outport  InitialOutput=0  VectorParamsAs1DForOutWhenUnconnected=off
  wires:
  n/1 -> FIMWB_144/1(Original)
  FIMWB_144/1(Result) -> a/1

== system all_sc_0001_0193/Subsystem/Layer Recurrent Neural Network 3 layers /Process Input 1/FIMWB_147 ==
  Original : Inport
  Result : Outport
  wires:
  Original/1 -> Result/1

== system all_sc_0001_0193/Subsystem/Layer Recurrent Neural Network 3 layers /Process Input 1/FIMWB_152 ==
  Original : Inport
  Result : Outport
  wires:
  Original/1 -> Result/1

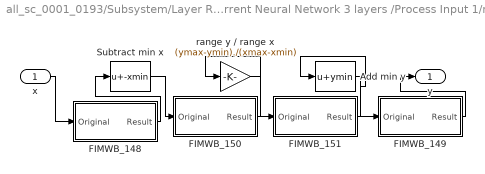
== system all_sc_0001_0193/Subsystem/Layer Recurrent Neural Network 3 layers /Process Input 1/mapminmax ==
  x : Inport
  Add min y : Bias  Bias=ymin  SaturateOnIntegerOverflow=off
  FIMWB_148 : Subsystem  Tag=fimwb.fault.148
  FIMWB_149 : Subsystem  Tag=fimwb.fault.149
  FIMWB_150 : Subsystem  Tag=fimwb.fault.150
  FIMWB_151 : Subsystem  Tag=fimwb.fault.151
  Subtract min x : Bias  Bias=-xmin  SaturateOnIntegerOverflow=off
  range y / range x : Gain  Gain=(ymax-ymin)./(xmax-xmin)
  y : Outport  VectorParamsAs1DForOutWhenUnconnected=off
  wires:
  x/1 -> FIMWB_148/1(Original)
  FIMWB_148/1(Result) -> Subtract min x/1
  Add min y/1 -> FIMWB_149/1(Original)
  FIMWB_149/1(Result) -> y/1
  Subtract min x/1 -> FIMWB_150/1(Original)
  FIMWB_150/1(Result) -> range y / range x/1
  range y / range x/1 -> FIMWB_151/1(Original)
  FIMWB_151/1(Result) -> Add min y/1

== system all_sc_0001_0193/Subsystem/Layer Recurrent Neural Network 3 layers /Process Output 1/FIMWB_154 ==
  Original : Inport
  Result : Outport
  wires:
  Original/1 -> Result/1

== system all_sc_0001_0193/Subsystem/Layer Recurrent Neural Network 3 layers /Process Output 1/FIMWB_159 ==
  Original : Inport
  Result : Outport
  wires:
  Original/1 -> Result/1

== system all_sc_0001_0193/Subsystem/Layer Recurrent Neural Network 3 layers /Process Output 1/mapminmax_reverse ==
  y : Inport
  Add min x : Bias  Bias=xmin  SaturateOnIntegerOverflow=off
  Divide by range y : Gain  Gain=(xmax-xmin)./(ymax-ymin)
  FIMWB_155 : Subsystem  Tag=fimwb.fault.155
  FIMWB_156 : Subsystem  Tag=fimwb.fault.156
  FIMWB_157 : Subsystem  Tag=fimwb.fault.157
  FIMWB_158 : Subsystem  Tag=fimwb.fault.158
  Subtract min y : Bias  Bias=-ymin  SaturateOnIntegerOverflow=off
  x : Outport  VectorParamsAs1DForOutWhenUnconnected=off
  wires:
  y/1 -> FIMWB_155/1(Original)
  FIMWB_155/1(Result) -> Subtract min y/1
  Add min x/1 -> FIMWB_156/1(Original)
  FIMWB_156/1(Result) -> x/1
  Divide by range y/1 -> FIMWB_157/1(Original)
  FIMWB_157/1(Result) -> Add min x/1
  Subtract min y/1 -> FIMWB_158/1(Original)
  FIMWB_158/1(Result) -> Divide by range y/1

== system all_sc_0001_0193/Subsystem/Steam Condenser1/Actuator/FIMWB_009 ==
  Original : Inport
  Result : Outport
  wires:
  Original/1 -> Result/1

== system all_sc_0001_0193/Subsystem/Steam Condenser1/Actuator/FIMWB_010 ==
  Original : Inport
  Result : Outport
  wires:
  Original/1 -> Result/1

== system all_sc_0001_0193/Subsystem/Steam Condenser1/sensor/FIMWB_042 ==
  Original : Inport
  Result : Outport
  wires:
  Original/1 -> Result/1

== system all_sc_0001_0193/Subsystem/Steam Condenser1/sensor/FIMWB_043 ==
  Original : Inport
  Result : Outport
  wires:
  Original/1 -> Result/1

== system all_sc_0001_0193/Subsystem/Layer Recurrent Neural Network 3 layers /Layer 1/Delays 1/FIMWB_058 ==
  Original : Inport
  Result : Outport
  wires:
  Original/1 -> Result/1

== system all_sc_0001_0193/Subsystem/Layer Recurrent Neural Network 3 layers /Layer 1/Delays 1/FIMWB_059 ==
  Original : Inport
  Result : Outport
  wires:
  Original/1 -> Result/1

== system all_sc_0001_0193/Subsystem/Layer Recurrent Neural Network 3 layers /Layer 1/Delays 2/FIMWB_061 ==
  Original : Inport
  Result : Outport
  wires:
  Original/1 -> Result/1

== system all_sc_0001_0193/Subsystem/Layer Recurrent Neural Network 3 layers /Layer 1/Delays 2/FIMWB_062 ==
  Original : Inport
  Result : Outport
  wires:
  Original/1 -> Result/1

== system all_sc_0001_0193/Subsystem/Layer Recurrent Neural Network 3 layers /Layer 1/Delays 2/FIMWB_063 ==
  Original : Inport
  Result : Outport
  wires:
  Original/1 -> Result/1

== system all_sc_0001_0193/Subsystem/Layer Recurrent Neural Network 3 layers /Layer 1/Delays 2/FIMWB_064 ==
  Original : Inport
  Result : Outport
  wires:
  Original/1 -> Result/1

== system all_sc_0001_0193/Subsystem/Layer Recurrent Neural Network 3 layers /Layer 1/Delays 2/FIMWB_065 ==
  Original : Inport
  Result : Outport
  wires:
  Original/1 -> Result/1

== system all_sc_0001_0193/Subsystem/Layer Recurrent Neural Network 3 layers /Layer 1/Delays 2/FIMWB_066 ==
  Original : Inport
  Result : Outport
  wires:
  Original/1 -> Result/1

== system all_sc_0001_0193/Subsystem/Layer Recurrent Neural Network 3 layers /Layer 1/Delays 2/FIMWB_067 ==
  Original : Inport
  Result : Outport
  wires:
  Original/1 -> Result/1

== system all_sc_0001_0193/Subsystem/Layer Recurrent Neural Network 3 layers /Layer 1/Delays 2/FIMWB_068 ==
  Original : Inport
  Result : Outport
  wires:
  Original/1 -> Result/1

== system all_sc_0001_0193/Subsystem/Layer Recurrent Neural Network 3 layers /Layer 1/Delays 2/FIMWB_069 ==
  Original : Inport
  Result : Outport
  wires:
  Original/1 -> Result/1

== system all_sc_0001_0193/Subsystem/Layer Recurrent Neural Network 3 layers /Layer 1/Delays 2/FIMWB_070 ==
  Original : Inport
  Result : Outport
  wires:
  Original/1 -> Result/1

== system all_sc_0001_0193/Subsystem/Layer Recurrent Neural Network 3 layers /Layer 1/Delays 2/FIMWB_071 ==
  Original : Inport
  Result : Outport
  wires:
  Original/1 -> Result/1

== system all_sc_0001_0193/Subsystem/Layer Recurrent Neural Network 3 layers /Layer 1/Delays 2/FIMWB_072 ==
  Original : Inport
  Result : Outport
  wires:
  Original/1 -> Result/1

== system all_sc_0001_0193/Subsystem/Layer Recurrent Neural Network 3 layers /Layer 1/Delays 2/FIMWB_073 ==
  Original : Inport
  Result : Outport
  wires:
  Original/1 -> Result/1

== system all_sc_0001_0193/Subsystem/Layer Recurrent Neural Network 3 layers /Layer 1/Delays 2/FIMWB_074 ==
  Original : Inport
  Result : Outport
  wires:
  Original/1 -> Result/1

== system all_sc_0001_0193/Subsystem/Layer Recurrent Neural Network 3 layers /Layer 1/Delays 2/FIMWB_075 ==
  Original : Inport
  Result : Outport
  wires:
  Original/1 -> Result/1

== system all_sc_0001_0193/Subsystem/Layer Recurrent Neural Network 3 layers /Layer 1/Delays 2/FIMWB_076 ==
  Original : Inport
  Result : Outport
  wires:
  Original/1 -> Result/1

== system all_sc_0001_0193/Subsystem/Layer Recurrent Neural Network 3 layers /Layer 1/Delays 2/FIMWB_188 ==
  Original : Inport
  Result : Outport
  wires:
  Original/1 -> Result/1

== system all_sc_0001_0193/Subsystem/Layer Recurrent Neural Network 3 layers /Layer 1/Delays 2/FIMWB_189 ==
  Original : Inport
  Result : Outport
  wires:
  Original/1 -> Result/1

== system all_sc_0001_0193/Subsystem/Layer Recurrent Neural Network 3 layers /Layer 1/Delays 2/FIMWB_190 ==
  Original : Inport
  Result : Outport
  wires:
  Original/1 -> Result/1

== system all_sc_0001_0193/Subsystem/Layer Recurrent Neural Network 3 layers /Layer 1/IW{1,1}/FIMWB_078 ==
  Original : Inport
  Result : Outport
  wires:
  Original/1 -> Result/1

== system all_sc_0001_0193/Subsystem/Layer Recurrent Neural Network 3 layers /Layer 1/IW{1,1}/FIMWB_079 ==
  Original : Inport
  Result : Outport
  wires:
  Original/1 -> Result/1

== system all_sc_0001_0193/Subsystem/Layer Recurrent Neural Network 3 layers /Layer 1/IW{1,1}/FIMWB_080 ==
  Original : Inport
  Result : Outport
  wires:
  Original/1 -> Result/1

== system all_sc_0001_0193/Subsystem/Layer Recurrent Neural Network 3 layers /Layer 1/IW{1,1}/FIMWB_081 ==
  Original : Inport
  Result : Outport
  wires:
  Original/1 -> Result/1

== system all_sc_0001_0193/Subsystem/Layer Recurrent Neural Network 3 layers /Layer 1/IW{1,1}/FIMWB_082 ==
  Original : Inport
  Result : Outport
  wires:
  Original/1 -> Result/1

== system all_sc_0001_0193/Subsystem/Layer Recurrent Neural Network 3 layers /Layer 1/IW{1,1}/FIMWB_083 ==
  Original : Inport
  Result : Outport
  wires:
  Original/1 -> Result/1

== system all_sc_0001_0193/Subsystem/Layer Recurrent Neural Network 3 layers /Layer 1/IW{1,1}/FIMWB_084 ==
  Original : Inport
  Result : Outport
  wires:
  Original/1 -> Result/1

== system all_sc_0001_0193/Subsystem/Layer Recurrent Neural Network 3 layers /Layer 1/IW{1,1}/FIMWB_088 ==
  Original : Inport
  Result : Outport
  wires:
  Original/1 -> Result/1

== system all_sc_0001_0193/Subsystem/Layer Recurrent Neural Network 3 layers /Layer 1/IW{1,1}/FIMWB_092 ==
  Original : Inport
  Result : Outport
  wires:
  Original/1 -> Result/1

== system all_sc_0001_0193/Subsystem/Layer Recurrent Neural Network 3 layers /Layer 1/IW{1,1}/FIMWB_096 ==
  Original : Inport
  Result : Outport
  wires:
  Original/1 -> Result/1

== system all_sc_0001_0193/Subsystem/Layer Recurrent Neural Network 3 layers /Layer 1/IW{1,1}/FIMWB_191 ==
  Original : Inport
  Result : Outport
  wires:
  Original/1 -> Result/1

== system all_sc_0001_0193/Subsystem/Layer Recurrent Neural Network 3 layers /Layer 1/IW{1,1}/dotprod1 ==
  In1 : Inport
  In2 : Inport  Port=2
  Dot Product : DotProduct  OutDataTypeStr=Inherit: Inherit via internal rule
  FIMWB_085 : Subsystem  Tag=fimwb.fault.85
  FIMWB_086 : Subsystem  Tag=fimwb.fault.86
  FIMWB_087 : Subsystem  Tag=fimwb.fault.87
  Out1 : Outport  VectorParamsAs1DForOutWhenUnconnected=off
  wires:
  In1/1 -> FIMWB_085/1(Original)
  FIMWB_085/1(Result) -> Dot Product/1
  In2/1 -> FIMWB_086/1(Original)
  FIMWB_086/1(Result) -> Dot Product/2
  Dot Product/1 -> FIMWB_087/1(Original)
  FIMWB_087/1(Result) -> Out1/1

== system all_sc_0001_0193/Subsystem/Layer Recurrent Neural Network 3 layers /Layer 1/IW{1,1}/dotprod2 ==
  In1 : Inport
  In2 : Inport  Port=2
  Dot Product : DotProduct  OutDataTypeStr=Inherit: Inherit via internal rule
  FIMWB_089 : Subsystem  Tag=fimwb.fault.89
  FIMWB_090 : Subsystem  Tag=fimwb.fault.90
  FIMWB_091 : Subsystem  Tag=fimwb.fault.91
  Out1 : Outport  VectorParamsAs1DForOutWhenUnconnected=off
  wires:
  In1/1 -> FIMWB_089/1(Original)
  FIMWB_089/1(Result) -> Dot Product/1
  In2/1 -> FIMWB_090/1(Original)
  FIMWB_090/1(Result) -> Dot Product/2
  Dot Product/1 -> FIMWB_091/1(Original)
  FIMWB_091/1(Result) -> Out1/1

== system all_sc_0001_0193/Subsystem/Layer Recurrent Neural Network 3 layers /Layer 1/IW{1,1}/dotprod3 ==
  In1 : Inport
  In2 : Inport  Port=2
  Dot Product : DotProduct  OutDataTypeStr=Inherit: Inherit via internal rule
  FIMWB_093 : Subsystem  Tag=fimwb.fault.93
  FIMWB_094 : Subsystem  Tag=fimwb.fault.94
  FIMWB_095 : Subsystem  Tag=fimwb.fault.95
  Out1 : Outport  VectorParamsAs1DForOutWhenUnconnected=off
  wires:
  In1/1 -> FIMWB_093/1(Original)
  FIMWB_093/1(Result) -> Dot Product/1
  In2/1 -> FIMWB_094/1(Original)
  FIMWB_094/1(Result) -> Dot Product/2
  Dot Product/1 -> FIMWB_095/1(Original)
  FIMWB_095/1(Result) -> Out1/1

== system all_sc_0001_0193/Subsystem/Layer Recurrent Neural Network 3 layers /Layer 1/LW{1,1}/FIMWB_098 ==
  Original : Inport
  Result : Outport
  wires:
  Original/1 -> Result/1

== system all_sc_0001_0193/Subsystem/Layer Recurrent Neural Network 3 layers /Layer 1/LW{1,1}/FIMWB_099 ==
  Original : Inport
  Result : Outport
  wires:
  Original/1 -> Result/1

== system all_sc_0001_0193/Subsystem/Layer Recurrent Neural Network 3 layers /Layer 1/LW{1,1}/FIMWB_100 ==
  Original : Inport
  Result : Outport
  wires:
  Original/1 -> Result/1

== system all_sc_0001_0193/Subsystem/Layer Recurrent Neural Network 3 layers /Layer 1/LW{1,1}/FIMWB_101 ==
  Original : Inport
  Result : Outport
  wires:
  Original/1 -> Result/1

== system all_sc_0001_0193/Subsystem/Layer Recurrent Neural Network 3 layers /Layer 1/LW{1,1}/FIMWB_102 ==
  Original : Inport
  Result : Outport
  wires:
  Original/1 -> Result/1

== system all_sc_0001_0193/Subsystem/Layer Recurrent Neural Network 3 layers /Layer 1/LW{1,1}/FIMWB_103 ==
  Original : Inport
  Result : Outport
  wires:
  Original/1 -> Result/1

== system all_sc_0001_0193/Subsystem/Layer Recurrent Neural Network 3 layers /Layer 1/LW{1,1}/FIMWB_104 ==
  Original : Inport
  Result : Outport
  wires:
  Original/1 -> Result/1

== system all_sc_0001_0193/Subsystem/Layer Recurrent Neural Network 3 layers /Layer 1/LW{1,1}/FIMWB_108 ==
  Original : Inport
  Result : Outport
  wires:
  Original/1 -> Result/1

== system all_sc_0001_0193/Subsystem/Layer Recurrent Neural Network 3 layers /Layer 1/LW{1,1}/FIMWB_112 ==
  Original : Inport
  Result : Outport
  wires:
  Original/1 -> Result/1

== system all_sc_0001_0193/Subsystem/Layer Recurrent Neural Network 3 layers /Layer 1/LW{1,1}/FIMWB_116 ==
  Original : Inport
  Result : Outport
  wires:
  Original/1 -> Result/1

== system all_sc_0001_0193/Subsystem/Layer Recurrent Neural Network 3 layers /Layer 1/LW{1,1}/FIMWB_192 ==
  Original : Inport
  Result : Outport
  wires:
  Original/1 -> Result/1

== system all_sc_0001_0193/Subsystem/Layer Recurrent Neural Network 3 layers /Layer 1/LW{1,1}/dotprod1 ==
  In1 : Inport
  In2 : Inport  Port=2
  Dot Product : DotProduct  OutDataTypeStr=Inherit: Inherit via internal rule
  FIMWB_105 : Subsystem  Tag=fimwb.fault.105
  FIMWB_106 : Subsystem  Tag=fimwb.fault.106
  FIMWB_107 : Subsystem  Tag=fimwb.fault.107
  Out1 : Outport  VectorParamsAs1DForOutWhenUnconnected=off
  wires:
  In1/1 -> FIMWB_105/1(Original)
  FIMWB_105/1(Result) -> Dot Product/1
  In2/1 -> FIMWB_106/1(Original)
  FIMWB_106/1(Result) -> Dot Product/2
  Dot Product/1 -> FIMWB_107/1(Original)
  FIMWB_107/1(Result) -> Out1/1

== system all_sc_0001_0193/Subsystem/Layer Recurrent Neural Network 3 layers /Layer 1/LW{1,1}/dotprod2 ==
  In1 : Inport
  In2 : Inport  Port=2
  Dot Product : DotProduct  OutDataTypeStr=Inherit: Inherit via internal rule
  FIMWB_109 : Subsystem  Tag=fimwb.fault.109
  FIMWB_110 : Subsystem  Tag=fimwb.fault.110
  FIMWB_111 : Subsystem  Tag=fimwb.fault.111
  Out1 : Outport  VectorParamsAs1DForOutWhenUnconnected=off
  wires:
  In1/1 -> FIMWB_109/1(Original)
  FIMWB_109/1(Result) -> Dot Product/1
  In2/1 -> FIMWB_110/1(Original)
  FIMWB_110/1(Result) -> Dot Product/2
  Dot Product/1 -> FIMWB_111/1(Original)
  FIMWB_111/1(Result) -> Out1/1

== system all_sc_0001_0193/Subsystem/Layer Recurrent Neural Network 3 layers /Layer 1/LW{1,1}/dotprod3 ==
  In1 : Inport
  In2 : Inport  Port=2
  Dot Product : DotProduct  OutDataTypeStr=Inherit: Inherit via internal rule
  FIMWB_113 : Subsystem  Tag=fimwb.fault.113
  FIMWB_114 : Subsystem  Tag=fimwb.fault.114
  FIMWB_115 : Subsystem  Tag=fimwb.fault.115
  Out1 : Outport  VectorParamsAs1DForOutWhenUnconnected=off
  wires:
  In1/1 -> FIMWB_113/1(Original)
  FIMWB_113/1(Result) -> Dot Product/1
  In2/1 -> FIMWB_114/1(Original)
  FIMWB_114/1(Result) -> Dot Product/2
  Dot Product/1 -> FIMWB_115/1(Original)
  FIMWB_115/1(Result) -> Out1/1

== system all_sc_0001_0193/Subsystem/Layer Recurrent Neural Network 3 layers /Layer 1/tansig/FIMWB_119 ==
  Original : Inport
  Result : Outport
  wires:
  Original/1 -> Result/1

== system all_sc_0001_0193/Subsystem/Layer Recurrent Neural Network 3 layers /Layer 1/tansig/FIMWB_120 ==
  Original : Inport
  Result : Outport
  wires:
  Original/1 -> Result/1

== system all_sc_0001_0193/Subsystem/Layer Recurrent Neural Network 3 layers /Layer 1/tansig/FIMWB_121 ==
  Original : Inport
  Result : Outport
  wires:
  Original/1 -> Result/1

== system all_sc_0001_0193/Subsystem/Layer Recurrent Neural Network 3 layers /Layer 1/tansig/FIMWB_122 ==
  Original : Inport
  Result : Outport
  wires:
  Original/1 -> Result/1

== system all_sc_0001_0193/Subsystem/Layer Recurrent Neural Network 3 layers /Layer 1/tansig/FIMWB_123 ==
  Original : Inport
  Result : Outport
  wires:
  Original/1 -> Result/1

== system all_sc_0001_0193/Subsystem/Layer Recurrent Neural Network 3 layers /Layer 1/tansig/FIMWB_124 ==
  Original : Inport
  Result : Outport
  wires:
  Original/1 -> Result/1

== system all_sc_0001_0193/Subsystem/Layer Recurrent Neural Network 3 layers /Layer 1/tansig/FIMWB_125 ==
  Original : Inport
  Result : Outport
  wires:
  Original/1 -> Result/1

== system all_sc_0001_0193/Subsystem/Layer Recurrent Neural Network 3 layers /Layer 1/tansig/FIMWB_126 ==
  Original : Inport
  Result : Outport
  wires:
  Original/1 -> Result/1

== system all_sc_0001_0193/Subsystem/Layer Recurrent Neural Network 3 layers /Layer 1/tansig/FIMWB_127 ==
  Original : Inport
  Result : Outport
  wires:
  Original/1 -> Result/1

== system all_sc_0001_0193/Subsystem/Layer Recurrent Neural Network 3 layers /Layer 2/Delays 1/FIMWB_132 ==
  Original : Inport
  Result : Outport
  wires:
  Original/1 -> Result/1
